simulink model "AFC_FFNN_trainscg_15_15_15_15_15_Nor_July_15_RepCont"  (R2021a)
settings: Solver=ode15s  StartTime=0.0  StopTime=T  MaxStep=.01  RelTol=1e-3
InitFcn:
  | ensure_patch_sig_in();
undefined symbols (not defined in the file): AF_sensor_tol, fault_time, fuel_inj_tol, kappa_tol, MAF_sensor_tol, pump_tol, tau_ww_tol, x_gain, x_offset, y_gain, y_offset
libraries: neural x82
(part 4 of 4)

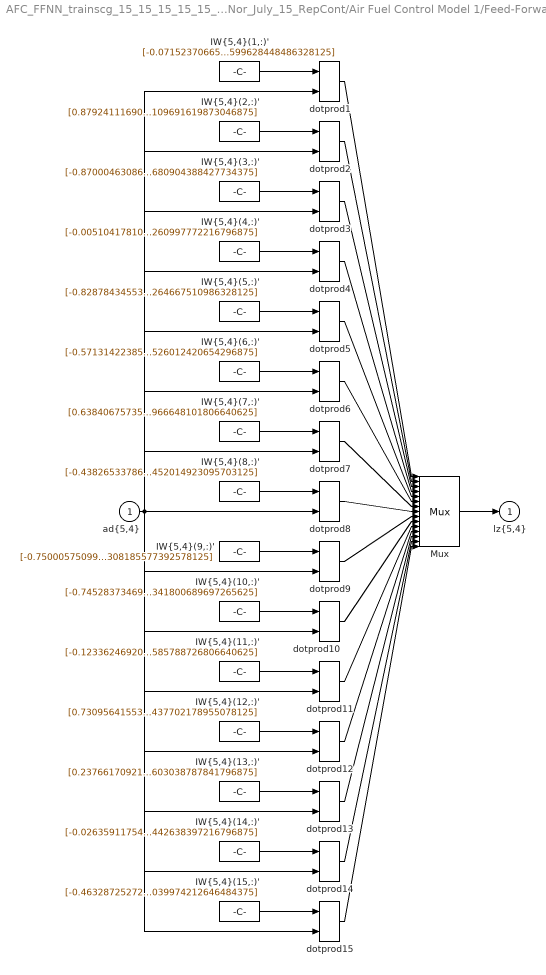
== system AFC_FFNN_trainscg_15_15_15_15_15_Nor_July_15_RepCont/Air Fuel Control Model 1/Feed-Forward Neural Network/Layer 5/LW{5,4} ==
  "ad{5,4}" : Inport  PortDimensions=15
      mask Display: e = 0.06;c1 = [120 230 180]/255;c2 = ([120 230 180]+0)/(256+128);c3 = ([120 230 180]+128)/(256+128);patch([0 1 1 0],[0 0 1 1],c1);patch([0 1 1 1-e 1-e 0+e],[0 0 1 1-e 0+e 0+e],c2);patch([0 0 1 1-e 0+e 0+e],[0 1 1 1-e 1-e 0+e],c3);plot([0 1 1 0 0],[0 0 1 1 0]);
  "IW{5,4}(1,:)'" : Constant  Value=[-0.0715237066501865637047075097143533639609813690185546875;-0.059455360452374352020488146308707655407488346099853515625;0.0042080898735644862995730619559253682382404804229736328125;0.2901089383986412695293211072566919028759002685546875;0.095073068854255371462613766198046505451202392578125;-0.7245204898788843994594799369224347174167633056640625;-0.95341156977462160337921659447601996362209320068359375;-0.381546919757219826774274906711070798337459564208984375;0.64062838445033254419769264131900854408740997314453125;-0.41532270884854227688265382312238216400146484375;0.9228342233845399089631200695293955504894256591796875;0.52678841002817666794300066612777300179004669189453125;0.92917047870120661468007483563269488513469696044921875;0.31486675897001215052029010621481575071811676025390625;0.0978604704135155600841500245223869569599628448486328125]
      mask Display: e = 0.06;c1 = [120 150 230]/255;c2 = ([120 150 230]+0)/383;c3 = ([120 150 230]+128)/383;patch([0 1 1 0],[0 0 1 1],c1);patch([0 1 1 1-e 1-e 0+e],[0 0 1 1-e 0+e 0+e],c2);patch([0 0 1 1-e 0+e 0+e],[0 1 1 1-e 1-e 0+e],c3);plot([0 1 1 0 0],[0 0 1 1 0]);disp('weights');
  "IW{5,4}(10,:)'" : Constant  Value=[-0.745283734691431387631155303097330033779144287109375;0.6327139929387517458536649428424425423145294189453125;0.1814176919217727335098544472202775068581104278564453125;0.44811074278119722436031224788166582584381103515625;-0.8904745653823924467218375866650603711605072021484375;-0.1411457300286087512830590640078298747539520263671875;0.6893492671787264658433969088946469128131866455078125;-0.92286808214381721438002159629832021892070770263671875;-0.702719569569371316219985601492226123809814453125;0.578347130669404574376812888658605515956878662109375;-0.433450867120990235292765646590851247310638427734375;-0.10595183853206820157044631969256442971527576446533203125;0.05814803339909381529881926553571247495710849761962890625;0.70409350150412330915372649542405270040035247802734375;0.49499370589664215547287540175602771341800689697265625]
      mask Display: e = 0.06;c1 = [120 150 230]/255;c2 = ([120 150 230]+0)/383;c3 = ([120 150 230]+128)/383;patch([0 1 1 0],[0 0 1 1],c1);patch([0 1 1 1-e 1-e 0+e],[0 0 1 1-e 0+e 0+e],c2);patch([0 0 1 1-e 0+e 0+e],[0 1 1 1-e 1-e 0+e],c3);plot([0 1 1 0 0],[0 0 1 1 0]);disp('weights');
  "IW{5,4}(11,:)'" : Constant  Value=[-0.1233624692016876689404369926705840043723583221435546875;0.7427858565377867261503297413582913577556610107421875;-0.6452270479684789616925399968749843537807464599609375;0.80229201087052237628682860304252244532108306884765625;-0.0568868193236429231518513915943913161754608154296875;0.6812541647223564478252910703304223716259002685546875;0.73478538636070300782421327312476933002471923828125;-0.90683981762392529279992459123604930937290191650390625;0.1533706191209432689870340027482598088681697845458984375;-0.2065977000624570347753206078778021037578582763671875;-0.69917607959227812131075552315451204776763916015625;0.26674758647147456258608144707977771759033203125;0.00914836505551542243652729524683309136889874935150146484375;-0.6399491125429499494003948711906559765338897705078125;0.0354412162674015152052930943682440556585788726806640625]
      mask Display: e = 0.06;c1 = [120 150 230]/255;c2 = ([120 150 230]+0)/383;c3 = ([120 150 230]+128)/383;patch([0 1 1 0],[0 0 1 1],c1);patch([0 1 1 1-e 1-e 0+e],[0 0 1 1-e 0+e 0+e],c2);patch([0 0 1 1-e 0+e 0+e],[0 1 1 1-e 1-e 0+e],c3);plot([0 1 1 0 0],[0 0 1 1 0]);disp('weights');
  "IW{5,4}(12,:)'" : Constant  Value=[0.73095641553966250736351639716303907334804534912109375;0.4871355339961243036128735184320248663425445556640625;-0.497421269660421050406995391313103027641773223876953125;0.797168206723321670637005809112451970577239990234375;0.417766150048340278999603469856083393096923828125;0.6564646990516640467916431589401327073574066162109375;0.7871861509157020986293673558975569903850555419921875;0.19888839208758846144320386883919127285480499267578125;0.83553010432982921518174634911702014505863189697265625;-0.411943496993746993695140190538950264453887939453125;0.922024497362436523673068222706206142902374267578125;0.518401102529268964502762173651717603206634521484375;-0.87560721497756077713603417578269727528095245361328125;0.57175513701463687166182126020430587232112884521484375;-0.8276073568365678312375166569836437702178955078125]
      mask Display: e = 0.06;c1 = [120 150 230]/255;c2 = ([120 150 230]+0)/383;c3 = ([120 150 230]+128)/383;patch([0 1 1 0],[0 0 1 1],c1);patch([0 1 1 1-e 1-e 0+e],[0 0 1 1-e 0+e 0+e],c2);patch([0 0 1 1-e 0+e 0+e],[0 1 1 1-e 1-e 0+e],c3);plot([0 1 1 0 0],[0 0 1 1 0]);disp('weights');
  "IW{5,4}(13,:)'" : Constant  Value=[0.2376617092170787426397282615653239190578460693359375;-0.9885705088057334943840714913676492869853973388671875;-0.886880268826178763674761285074055194854736328125;0.7061210321519670873868790295091457664966583251953125;-0.6273662474377628139876605928293429315090179443359375;-0.998268267412152798812030596309341490268707275390625;-0.4703689472235585977699656723416410386562347412109375;-0.9241992366964633109915894237929023802280426025390625;-0.747719904959309733527561547816731035709381103515625;0.8818924664208236396945039814454503357410430908203125;0.07674704745712279674307865207083523273468017578125;-0.4112203622036787464821827597916126251220703125;0.83385659205751228029157573473639786243438720703125;-0.25162142736245396434924259665422141551971435546875;-0.180344219235205827089885133318603038787841796875]
      mask Display: e = 0.06;c1 = [120 150 230]/255;c2 = ([120 150 230]+0)/383;c3 = ([120 150 230]+128)/383;patch([0 1 1 0],[0 0 1 1],c1);patch([0 1 1 1-e 1-e 0+e],[0 0 1 1-e 0+e 0+e],c2);patch([0 0 1 1-e 0+e 0+e],[0 1 1 1-e 1-e 0+e],c3);plot([0 1 1 0 0],[0 0 1 1 0]);disp('weights');
  "IW{5,4}(14,:)'" : Constant  Value=[-0.0263591175497553918682935858441851451061666011810302734375;-0.73862473877419976275859880843199789524078369140625;-0.9818407470620658106241762652643956243991851806640625;-0.8322907510546138087903500490938313305377960205078125;-0.40775753473065368126526664127595722675323486328125;0.85727737303545215041822302737273275852203369140625;-0.913714783630615645648731515393592417240142822265625;-0.434025787294483100797748420518473722040653228759765625;0.51057369949210862358768281410448253154754638671875;-0.923275801188926603657591840601526200771331787109375;-0.6364652652927833553775371910887770354747772216796875;0.7604639939080046762143183514126576483249664306640625;0.559391998498745213197480552480556070804595947265625;0.51465198508545284550308451798628084361553192138671875;0.40409177873949164716549375953036360442638397216796875]
      mask Display: e = 0.06;c1 = [120 150 230]/255;c2 = ([120 150 230]+0)/383;c3 = ([120 150 230]+128)/383;patch([0 1 1 0],[0 0 1 1],c1);patch([0 1 1 1-e 1-e 0+e],[0 0 1 1-e 0+e 0+e],c2);patch([0 0 1 1-e 0+e 0+e],[0 1 1 1-e 1-e 0+e],c3);plot([0 1 1 0 0],[0 0 1 1 0]);disp('weights');
  "IW{5,4}(15,:)'" : Constant  Value=[-0.46328725272275139701605439768172800540924072265625;-0.141458750541851419058048122678883373737335205078125;0.417359177593134678119213276659138500690460205078125;-0.7778940511957792569575076413457281887531280517578125;-0.274320322427507701235072090639732778072357177734375;-0.7019314613676590486335271634743548929691314697265625;-0.7879876969556496302260484299040399491786956787109375;0.7965061683491236887988407033844850957393646240234375;0.2892567451407488388070987639366649091243743896484375;-0.805571707848603768553630288806743919849395751953125;-0.163626497462990183606734717614017426967620849609375;-0.683466400463462964154359724489040672779083251953125;-0.2210723476022076194880128241493366658687591552734375;-0.8756542550710353367549032554961740970611572265625;-0.0916336575431715427697554332553409039974212646484375]
      mask Display: e = 0.06;c1 = [120 150 230]/255;c2 = ([120 150 230]+0)/383;c3 = ([120 150 230]+128)/383;patch([0 1 1 0],[0 0 1 1],c1);patch([0 1 1 1-e 1-e 0+e],[0 0 1 1-e 0+e 0+e],c2);patch([0 0 1 1-e 0+e 0+e],[0 1 1 1-e 1-e 0+e],c3);plot([0 1 1 0 0],[0 0 1 1 0]);disp('weights');
  "IW{5,4}(2,:)'" : Constant  Value=[0.8792411169036473683746635288116522133350372314453125;0.9476643750844193636595491625485010445117950439453125;-0.121014662404281547747331160280737094581127166748046875;-0.64955468710774566520882444820017553865909576416015625;-0.2192888029702277918886466068215668201446533203125;0.9482089460418883231085374063695780932903289794921875;0.81071456577514011687668471495271660387516021728515625;-0.8778539344975506697466016703401692211627960205078125;-0.5367666595045050836887412515352480113506317138671875;-0.0818759946323519560706927222781814634799957275390625;-0.00147913782462527620964465313591063022613525390625;0.97707803825832273414420114931999705731868743896484375;-0.57967360625535724327761499807820655405521392822265625;0.7041045664752501043182064677239395678043365478515625;-0.71981214912070068390193000595900230109691619873046875]
      mask Display: e = 0.06;c1 = [120 150 230]/255;c2 = ([120 150 230]+0)/383;c3 = ([120 150 230]+128)/383;patch([0 1 1 0],[0 0 1 1],c1);patch([0 1 1 1-e 1-e 0+e],[0 0 1 1-e 0+e 0+e],c2);patch([0 0 1 1-e 0+e 0+e],[0 1 1 1-e 1-e 0+e],c3);plot([0 1 1 0 0],[0 0 1 1 0]);disp('weights');
  "IW{5,4}(3,:)'" : Constant  Value=[-0.870004630865640837811270102974958717823028564453125;-0.1394130191014479880351473184418864548206329345703125;0.44929842102961747851708196321851573884487152099609375;0.9390056072431598455096946054254658520221710205078125;0.3392077142091143304725164853152818977832794189453125;0.2638263459878500416522228988469578325748443603515625;-0.1271702216377524063961601541450363583862781524658203125;0.824871971464007369689852566807530820369720458984375;0.752978288612214274877487696358002722263336181640625;-0.358871719956378232296856367611326277256011962890625;0.3877730536909573810788742775912396609783172607421875;-0.1622420881467621089910835507907904684543609619140625;0.23014593691751572546166926258592866361141204833984375;-0.88941897035361938694819627926335670053958892822265625;-0.74207495222659980438351112752570770680904388427734375]
      mask Display: e = 0.06;c1 = [120 150 230]/255;c2 = ([120 150 230]+0)/383;c3 = ([120 150 230]+128)/383;patch([0 1 1 0],[0 0 1 1],c1);patch([0 1 1 1-e 1-e 0+e],[0 0 1 1-e 0+e 0+e],c2);patch([0 0 1 1-e 0+e 0+e],[0 1 1 1-e 1-e 0+e],c3);plot([0 1 1 0 0],[0 0 1 1 0]);disp('weights');
  "IW{5,4}(4,:)'" : Constant  Value=[-0.005104178107196749754337350424293617834337055683135986328125;0.723242918597417627779577742330729961395263671875;0.1777800728242972805315247342150541953742504119873046875;-0.2315142766680377828247827665109070949256420135498046875;0.66432988641756995917830863618291914463043212890625;-0.4486087512464720372662441150168888270854949951171875;-0.96268451305722180233459539522300474345684051513671875;-0.5291219806882916376622461029910482466220855712890625;-0.6246384153151449680763107608072459697723388671875;-0.7168661734093217940966269452474080026149749755859375;0.163315871632827569470691742026247084140777587890625;-0.6104447643185764160733697281102649867534637451171875;0.58602976789892957665273343081935308873653411865234375;0.88462651353997456826760981130064465105533599853515625;0.2406072415787565699218930603819899260997772216796875]
      mask Display: e = 0.06;c1 = [120 150 230]/255;c2 = ([120 150 230]+0)/383;c3 = ([120 150 230]+128)/383;patch([0 1 1 0],[0 0 1 1],c1);patch([0 1 1 1-e 1-e 0+e],[0 0 1 1-e 0+e 0+e],c2);patch([0 0 1 1-e 0+e 0+e],[0 1 1 1-e 1-e 0+e],c3);plot([0 1 1 0 0],[0 0 1 1 0]);disp('weights');
  "IW{5,4}(5,:)'" : Constant  Value=[-0.8287843455345054177740848899702541530132293701171875;0.60702538017370255563065484238904900848865509033203125;-0.19355408020178421768520138357416726648807525634765625;0.8884086963255166669028994874679483473300933837890625;0.02810771528634337101948403869755566120147705078125;-0.05301070772614746573481170344166457653045654296875;-0.65137729229106067219134956758352927863597869873046875;0.4202804667444233199802283706958405673503875732421875;-0.57904508252670738865930388783453963696956634521484375;0.5686244136944262894672874608659185469150543212890625;-0.328574866563430934007783434935845434665679931640625;0.0905545868520955254954429847202845849096775054931640625;-0.349451482700606330666914800531230866909027099609375;0.042456016757196547717345680439393618144094944000244140625;0.1761051545277756702478910710851778276264667510986328125]
      mask Display: e = 0.06;c1 = [120 150 230]/255;c2 = ([120 150 230]+0)/383;c3 = ([120 150 230]+128)/383;patch([0 1 1 0],[0 0 1 1],c1);patch([0 1 1 1-e 1-e 0+e],[0 0 1 1-e 0+e 0+e],c2);patch([0 0 1 1-e 0+e 0+e],[0 1 1 1-e 1-e 0+e],c3);plot([0 1 1 0 0],[0 0 1 1 0]);disp('weights');
  "IW{5,4}(6,:)'" : Constant  Value=[-0.5713142238533446271020466156187467277050018310546875;-0.503576738999999662382833776064217090606689453125;-0.6481484936093604432016945793293416500091552734375;-0.1183454483920598765411824615512159653007984161376953125;0.8834983524723070136275282493443228304386138916015625;-0.7475172422529510196653745879302732646465301513671875;-1.0046336664456265719280736448126845061779022216796875;0.608725088947579706655233167111873626708984375;0.499049521527679729171467215564916841685771942138671875;0.52599052748356456277178949676454067230224609375;0.2859724590846799419097123973187990486621856689453125;-0.75506229605684749284222334608784876763820648193359375;-0.384006528183055750869101530042826198041439056396484375;0.59518858313426858952510656308731995522975921630859375;-0.3364401719934875245598959736526012420654296875]
      mask Display: e = 0.06;c1 = [120 150 230]/255;c2 = ([120 150 230]+0)/383;c3 = ([120 150 230]+128)/383;patch([0 1 1 0],[0 0 1 1],c1);patch([0 1 1 1-e 1-e 0+e],[0 0 1 1-e 0+e 0+e],c2);patch([0 0 1 1-e 0+e 0+e],[0 1 1 1-e 1-e 0+e],c3);plot([0 1 1 0 0],[0 0 1 1 0]);disp('weights');
  "IW{5,4}(7,:)'" : Constant  Value=[0.6384067573591323263570984636317007243633270263671875;-0.398906189376702524640450064907781779766082763671875;0.3590663490432792759321500852820463478565216064453125;0.9824522582283503613354014305514283478260040283203125;-0.1817236106276645113410950216348282992839813232421875;0.33684980648238660450033421511761844158172607421875;-0.63399701385133511166714015416800975799560546875;-0.7621407404871585189454208375536836683750152587890625;-0.8769903337800799558721109860925935208797454833984375;-0.4675323855823581009616418668883852660655975341796875;-0.805696629997617375096297109848819673061370849609375;-0.4819410402133545989755702976253814995288848876953125;0.496426452433425868804306446691043674945831298828125;-0.51429089900277258351479758857749402523040771484375;-0.3450216144076565516485288753756321966648101806640625]
      mask Display: e = 0.06;c1 = [120 150 230]/255;c2 = ([120 150 230]+0)/383;c3 = ([120 150 230]+128)/383;patch([0 1 1 0],[0 0 1 1],c1);patch([0 1 1 1-e 1-e 0+e],[0 0 1 1-e 0+e 0+e],c2);patch([0 0 1 1-e 0+e 0+e],[0 1 1 1-e 1-e 0+e],c3);plot([0 1 1 0 0],[0 0 1 1 0]);disp('weights');
  "IW{5,4}(8,:)'" : Constant  Value=[-0.43826533786090704492011127513251267373561859130859375;-0.177428161616140556144927131754229776561260223388671875;-0.55432434021778254074064307133085094392299652099609375;0.1574437223343636838013281931125675328075885772705078125;0.4222152666047025437734419028856791555881500244140625;0.669107579605679791967531855334527790546417236328125;-0.89015338475136795981512705111526884138584136962890625;-0.81263781446701732757986746946698985993862152099609375;-0.73447676533593952985512487430241890251636505126953125;-0.881409950336343950283435333403758704662322998046875;0.5306763737125665958416220746585167944431304931640625;-0.258124212915001260970626617563539184629917144775390625;0.60220637617682515330130854636081494390964508056640625;0.59081506636078129357514399089268408715724945068359375;0.5258786458552944242939020114135928452014923095703125]
      mask Display: e = 0.06;c1 = [120 150 230]/255;c2 = ([120 150 230]+0)/383;c3 = ([120 150 230]+128)/383;patch([0 1 1 0],[0 0 1 1],c1);patch([0 1 1 1-e 1-e 0+e],[0 0 1 1-e 0+e 0+e],c2);patch([0 0 1 1-e 0+e 0+e],[0 1 1 1-e 1-e 0+e],c3);plot([0 1 1 0 0],[0 0 1 1 0]);disp('weights');
  "IW{5,4}(9,:)'" : Constant  Value=[-0.75000575099870292472559185625868849456310272216796875;0.79529760800211957150196440125000663101673126220703125;0.6376047718358714977426870973431505262851715087890625;-0.483394652199553409577248430650797672569751739501953125;0.103791975354226462258111496339552104473114013671875;-0.471845248230328362382124396390281617641448974609375;0.394311694379341604044242330928682349622249603271484375;0.26681610727024551721342504606582224369049072265625;0.84738192844972914929968510477920062839984893798828125;0.2339243378057733746544499808805994689464569091796875;0.8609789815849964167426833228091709315776824951171875;0.9634103237621685078551081460318528115749359130859375;0.191715289750559458870071694036596454679965972900390625;-0.29679487907828738801896406585001386702060699462890625;0.8576116780544318363155298357014544308185577392578125]
      mask Display: e = 0.06;c1 = [120 150 230]/255;c2 = ([120 150 230]+0)/383;c3 = ([120 150 230]+128)/383;patch([0 1 1 0],[0 0 1 1],c1);patch([0 1 1 1-e 1-e 0+e],[0 0 1 1-e 0+e 0+e],c2);patch([0 0 1 1-e 0+e 0+e],[0 1 1 1-e 1-e 0+e],c3);plot([0 1 1 0 0],[0 0 1 1 0]);disp('weights');
  Mux : Mux  Inputs=15
      mask Display: e = 0.06;c1 = [120 150 230]/255;c2 = ([120 150 230]+0)/383;c3 = ([120 150 230]+128)/383;patch([0 1 1 0],[0 0 1 1],c1);patch([0 1 1 1-e 1-e 0+e],[0 0 1 1-e 0+e 0+e],c2);patch([0 0 1 1-e 0+e 0+e],[0 1 1 1-e 1-e 0+e],c3);plot([0 1 1 0 0],[0 0 1 1 0]);disp('Mux');
  dotprod{1..15} (15 alike) : neural/Weight Functions/dotprod
  "lz{5,4}" : Outport
      mask Display: e = 0.06;c1 = [120 230 180]/255;c2 = ([120 230 180]+0)/(256+128);c3 = ([120 230 180]+128)/(256+128);patch([0 1 1 0],[0 0 1 1],c1);patch([0 1 1 1-e 1-e 0+e],[0 0 1 1-e 0+e 0+e],c2);patch([0 0 1 1-e 0+e 0+e],[0 1 1 1-e 1-e 0+e],c3);plot([0 1 1 0 0],[0 0 1 1 0]);
  wires:
  Mux/1 -> "lz{5,4}"/1
  dotprod15/1 -> Mux/15
  "IW{5,4}(15,:)'"/1 -> dotprod15/1
  dotprod14/1 -> Mux/14
  "IW{5,4}(14,:)'"/1 -> dotprod14/1
  dotprod13/1 -> Mux/13
  "IW{5,4}(13,:)'"/1 -> dotprod13/1
  dotprod12/1 -> Mux/12
  "IW{5,4}(12,:)'"/1 -> dotprod12/1
  dotprod11/1 -> Mux/11
  "IW{5,4}(11,:)'"/1 -> dotprod11/1
  dotprod10/1 -> Mux/10
  "IW{5,4}(10,:)'"/1 -> dotprod10/1
  dotprod9/1 -> Mux/9
  "IW{5,4}(9,:)'"/1 -> dotprod9/1
  dotprod8/1 -> Mux/8
  "IW{5,4}(8,:)'"/1 -> dotprod8/1
  dotprod7/1 -> Mux/7
  "IW{5,4}(7,:)'"/1 -> dotprod7/1
  dotprod6/1 -> Mux/6
  "IW{5,4}(6,:)'"/1 -> dotprod6/1
  dotprod5/1 -> Mux/5
  "IW{5,4}(5,:)'"/1 -> dotprod5/1
  dotprod4/1 -> Mux/4
  "IW{5,4}(4,:)'"/1 -> dotprod4/1
  dotprod3/1 -> Mux/3
  "IW{5,4}(3,:)'"/1 -> dotprod3/1
  dotprod2/1 -> Mux/2
  "IW{5,4}(2,:)'"/1 -> dotprod2/1
  dotprod1/1 -> Mux/1
  "ad{5,4}"/1 -> dotprod15/2, dotprod14/2, dotprod13/2, dotprod12/2, dotprod11/2, dotprod10/2, dotprod9/2, dotprod8/2, dotprod7/2, dotprod6/2, dotprod5/2, dotprod4/2, dotprod3/2, dotprod2/2, dotprod1/2
  "IW{5,4}(1,:)'"/1 -> dotprod1/1

== system AFC_FFNN_trainscg_15_15_15_15_15_Nor_July_15_RepCont/Air Fuel Control Model 1/Feed-Forward Neural Network/Layer 6/Delays 1 ==
  "p{6}" : Inport  PortDimensions=15
      mask Display: e = 0.06;c1 = [120 230 180]/255;c2 = ([120 230 180]+0)/(256+128);c3 = ([120 230 180]+128)/(256+128);patch([0 1 1 0],[0 0 1 1],c1);patch([0 1 1 1-e 1-e 0+e],[0 0 1 1-e 0+e 0+e],c2);patch([0 0 1 1-e 0+e 0+e],[0 1 1 1-e 1-e 0+e],c3);plot([0 1 1 0 0],[0 0 1 1 0]);
  mux : Mux  Inputs=1
      mask Display: e = 0.06;c1 = [120 150 230]/255;c2 = ([120 150 230]+0)/383;c3 = ([120 150 230]+128)/383;patch([0 1 1 0],[0 0 1 1],c1);patch([0 1 1 1-e 1-e 0+e],[0 0 1 1-e 0+e 0+e],c2);patch([0 0 1 1-e 0+e 0+e],[0 1 1 1-e 1-e 0+e],c3);plot([0 1 1 0 0],[0 0 1 1 0]);disp('Mux')
  "pd{6,5}" : Outport
      mask Display: e = 0.06;c1 = [120 230 180]/255;c2 = ([120 230 180]+0)/(256+128);c3 = ([120 230 180]+128)/(256+128);patch([0 1 1 0],[0 0 1 1],c1);patch([0 1 1 1-e 1-e 0+e],[0 0 1 1-e 0+e 0+e],c2);patch([0 0 1 1-e 0+e 0+e],[0 1 1 1-e 1-e 0+e],c3);plot([0 1 1 0 0],[0 0 1 1 0]);
  wires:
  mux/1 -> "pd{6,5}"/1
  "p{6}"/1 -> mux/1

== system AFC_FFNN_trainscg_15_15_15_15_15_Nor_July_15_RepCont/Air Fuel Control Model 1/Feed-Forward Neural Network/Layer 6/LW{6,5} ==
  "ad{6,5}" : Inport  PortDimensions=15
      mask Display: e = 0.06;c1 = [120 230 180]/255;c2 = ([120 230 180]+0)/(256+128);c3 = ([120 230 180]+128)/(256+128);patch([0 1 1 0],[0 0 1 1],c1);patch([0 1 1 1-e 1-e 0+e],[0 0 1 1-e 0+e 0+e],c2);patch([0 0 1 1-e 0+e 0+e],[0 1 1 1-e 1-e 0+e],c3);plot([0 1 1 0 0],[0 0 1 1 0]);
  "IW{6,5}(1,:)'" : Constant  Value=[-0.123794355159188906867484547547064721584320068359375;-0.54342989784435513644922366438549943268299102783203125;0.67191439248000695005913485147175379097461700439453125;-0.52498234414585687179766182453022338449954986572265625;-0.467335260607861291415332516407943330705165863037109375;-0.199615927195639308866503824901883490383625030517578125;0.21435004773181720594266153057105839252471923828125;0.91169194707349332507106964840204454958438873291015625;0.02540510237598773979339483730655047111213207244873046875;0.63533396914472561878284295744379051029682159423828125;-0.1332576588371870152105458373625879175961017608642578125;-0.57005408254605860474129030990297906100749969482421875;-0.0886450937949223582990043723839335143566131591796875;0.36612079421426901859604186029173433780670166015625;-0.1895090319374348464265267466544173657894134521484375]
      mask Display: e = 0.06;c1 = [120 150 230]/255;c2 = ([120 150 230]+0)/383;c3 = ([120 150 230]+128)/383;patch([0 1 1 0],[0 0 1 1],c1);patch([0 1 1 1-e 1-e 0+e],[0 0 1 1-e 0+e 0+e],c2);patch([0 0 1 1-e 0+e 0+e],[0 1 1 1-e 1-e 0+e],c3);plot([0 1 1 0 0],[0 0 1 1 0]);disp('weights');
  Mux : Mux  Inputs=1
      mask Display: e = 0.06;c1 = [120 150 230]/255;c2 = ([120 150 230]+0)/383;c3 = ([120 150 230]+128)/383;patch([0 1 1 0],[0 0 1 1],c1);patch([0 1 1 1-e 1-e 0+e],[0 0 1 1-e 0+e 0+e],c2);patch([0 0 1 1-e 0+e 0+e],[0 1 1 1-e 1-e 0+e],c3);plot([0 1 1 0 0],[0 0 1 1 0]);disp('Mux');
  dotprod1 : neural/Weight Functions/dotprod
  "lz{6,5}" : Outport
      mask Display: e = 0.06;c1 = [120 230 180]/255;c2 = ([120 230 180]+0)/(256+128);c3 = ([120 230 180]+128)/(256+128);patch([0 1 1 0],[0 0 1 1],c1);patch([0 1 1 1-e 1-e 0+e],[0 0 1 1-e 0+e 0+e],c2);patch([0 0 1 1-e 0+e 0+e],[0 1 1 1-e 1-e 0+e],c3);plot([0 1 1 0 0],[0 0 1 1 0]);
  wires:
  Mux/1 -> "lz{6,5}"/1
  dotprod1/1 -> Mux/1
  "ad{6,5}"/1 -> dotprod1/2
  "IW{6,5}(1,:)'"/1 -> dotprod1/1
